simulink model "ASM_Traffic"  (R2026a)
settings: Solver=ode1  StartTime=SIM.tstart.v  StopTime=SIM.tend.v  FixedStep=SIM.StepSize.v
PostLoadFcn:
  | if any(exist('dsrtsu_mdlpostloadfcn', 'file') ~= 0), dsrtsu_mdlpostloadfcn('Execute', bdroot); end
  | try, asm_mdl_postloadfcn(bdroot, 'UpdateModel', 3600); catch, disp(lasterr); end,
InitFcn:
  | , if any(exist('rtifpga_mdlclblib', 'file') ~= 0), rtifpga_mdlclblib('Init', bdroot); end,
  | , if any(exist('dsmpb_private', 'file') ~= 0), dsmpb_private('dsmpb_mdlclblib', 'Init', bdroot); end,
model workspace (MAT data in the model file):
  asmReferencePath = [0 0.01 0.02 0.03 0.04 0.05 0.06 0.07 0.08 0.09 0.1 0.11 ... (350007 elements, 50001x7)]
  roadBounds : Simulink.Parameter (value not decoded)
  safetyAxes : Simulink.Parameter (value not decoded)
undefined symbols (not defined in the file): _to_, a0b2, ASM_BrakeHydraulics_DemoSystems, ASM_VehicleDynamics_DemoSystems, b98103fe8ad365046cd0, BrakeCircuit, controllerConfig, CPT, Crankshaft, DiscIntNeverNeededParam, dsmsi, FinalDriveAssembly, MDL, ModeSignals, mu, Pos_BrakePedal_Maneuver, rad, RefSignals, roadFamilyData, roadFamilyId, s_to_rpm, SIM, SoftECU, Suspension, Tire, Transmission
libraries: ASM_Traffic_lib x135, simulink x98, ASM_Utils_lib x77, ASM_VehicleDynamics_lib x70, ASM_Environment_lib x22, dsmpblib x20, dsmsilib x15, MDLD_Utils_lib x10, ASM_BrakeHydraulics_lib x3, sl_discontinuities x2
(part 28 of 65)

== system ASM_Traffic/Environment/Road/PlantModel/Pos_CP_CoorsSys_E[:][x;y][m] ==
  Pos_CP[x;y][m] : Inport
  Active_CP_VehDyn_Trailer[] : Inport  Port=2
  Bus Selector : BusSelector  OutputSignals=Pos_CP_FL_CoorSys_E[x;y][m],Pos_CP_FR_CoorSys_E[x;y][m],Pos_CP_RL_CoorSys_E[x;y][m],Pos_CP_RL2_CoorSys_E[x;y][m],Pos_CP_RR_CoorSys_E[x;y][m],Pos_CP_RR2_CoorSys_E[x;y][m],Pos_CP_R2L_CoorSys_E[x;y][m],Pos_CP_R2L2_CoorSys_E[x;y][m],Pos_CP_R2R_CoorSys_E[x;y][m],Pos_CP_R2R2_CoorSys_E[x;y][m],Pos_CP_FL_Trailer_CoorSys_E[x;y][m],Pos_CP_FL2_Trailer_CoorSys_E[x;y][m],Pos_CP_FR_Trailer_CoorSys_E[x;y][m],Pos_CP_FR2_Trailer_CoorSys_E[x;y][m],Pos_CP_RL_Trailer_CoorSys_E[x;y][m],Pos_CP_RL2_Trailer_CoorSys_E[x;y][m],Pos_CP_RR_Trailer_CoorSys_E[x;y][m],Pos_CP_RR2_Trailer_CoorSys_E[x;y][m],Pos_CP_R2L_Trailer_CoorSys_E[x;y][m],Pos_CP_R2L2_Trailer_CoorSys_E[x;y][m],Pos_CP_R2R_Trailer_CoorSys_E[x;y][m],Pos_CP_R2R2_Trailer_CoorSys_E[x;y][m],Pos_CP_Front_CoorSys_E[x;y][m],Pos_CP_Rear_CoorSys_E[x;y][m]
  Mux : Mux  Inputs=24
  Selector : Selector  IndexOptions=Index vector (port)  Indices=[1 3]  OutputSizes=1
  Pos_CP_CoorsSys_E[:][x;y][m] : Outport  VectorParamsAs1DForOutWhenUnconnected=off
  wires:
  Bus Selector/24 -> Mux/24  "<Pos_CP_Rear_CoorSys_E[x;y][m]>"
  Bus Selector/23 -> Mux/23  "<Pos_CP_Front_CoorSys_E[x;y][m]>"
  Selector/1 -> Pos_CP_CoorsSys_E[:][x;y][m]/1
  Active_CP_VehDyn_Trailer[]/1 -> Selector/2
  Pos_CP[x;y][m]/1 -> Bus Selector/1
  Bus Selector/1 -> Mux/1  "<Pos_CP_FL_CoorSys_E[x;y][m]>"
  Bus Selector/2 -> Mux/2  "<Pos_CP_FR_CoorSys_E[x;y][m]>"
  Bus Selector/3 -> Mux/3  "<Pos_CP_RL_CoorSys_E[x;y][m]>"
  Bus Selector/4 -> Mux/4  "<Pos_CP_RL2_CoorSys_E[x;y][m]>"
  Bus Selector/5 -> Mux/5  "<Pos_CP_RR_CoorSys_E[x;y][m]>"
  Bus Selector/6 -> Mux/6  "<Pos_CP_RR2_CoorSys_E[x;y][m]>"
  Bus Selector/7 -> Mux/7  "<Pos_CP_R2L_CoorSys_E[x;y][m]>"
  Bus Selector/8 -> Mux/8  "<Pos_CP_R2L2_CoorSys_E[x;y][m]>"
  Bus Selector/9 -> Mux/9  "<Pos_CP_R2R_CoorSys_E[x;y][m]>"
  Bus Selector/10 -> Mux/10  "<Pos_CP_R2R2_CoorSys_E[x;y][m]>"
  Bus Selector/11 -> Mux/11  "<Pos_CP_FL_Trailer_CoorSys_E[x;y][m]>"
  Bus Selector/12 -> Mux/12  "<Pos_CP_FL2_Trailer_CoorSys_E[x;y][m]>"
  Bus Selector/13 -> Mux/13  "<Pos_CP_FR_Trailer_CoorSys_E[x;y][m]>"
  Bus Selector/14 -> Mux/14  "<Pos_CP_FR2_Trailer_CoorSys_E[x;y][m]>"
  Bus Selector/15 -> Mux/15  "<Pos_CP_RL_Trailer_CoorSys_E[x;y][m]>"
  Bus Selector/16 -> Mux/16  "<Pos_CP_RL2_Trailer_CoorSys_E[x;y][m]>"
  Bus Selector/17 -> Mux/17  "<Pos_CP_RR_Trailer_CoorSys_E[x;y][m]>"
  Bus Selector/18 -> Mux/18  "<Pos_CP_RR2_Trailer_CoorSys_E[x;y][m]>"
  Bus Selector/19 -> Mux/19  "<Pos_CP_R2L_Trailer_CoorSys_E[x;y][m]>"
  Bus Selector/20 -> Mux/20  "<Pos_CP_R2L2_Trailer_CoorSys_E[x;y][m]>"
  Bus Selector/21 -> Mux/21  "<Pos_CP_R2R_Trailer_CoorSys_E[x;y][m]>"
  Bus Selector/22 -> Mux/22  "<Pos_CP_R2R2_Trailer_CoorSys_E[x;y][m]>"
  Mux/1 -> Selector/1

== system ASM_Traffic/Environment/Road/PlantModel/Reload_Trigger ==
  Init_External_Additional[0Off|1On] : Inport
  Interface_Mode[0Off|1ObjectsOnly|2ObjectsAndLanes] : Inport  Port=2
  Constant3 : Constant  Value=0.5
  Constant5 : Constant
  Constant6 : Constant  Value=0
  Logical Operator1 : Logic  AllPortsSameDT=off
  Relational Operator2 : RelationalOperator  Operator=>  OutDataTypeStr=boolean  InputSameDT=off
  Start : MultiPortSwitch  DataPortOrder=Zero-based contiguous  Inputs=2  zeroidx=on  InputSameDT=off
  Ctrl_Reload[] : Outport  VectorParamsAs1DForOutWhenUnconnected=off
  wires:
  Relational Operator2/1 -> Logical Operator1/1
  Constant3/1 -> Relational Operator2/2
  Init_External_Additional[0Off|1On]/1 -> Logical Operator1/2
  Logical Operator1/1 -> Start/1
  Interface_Mode[0Off|1ObjectsOnly|2ObjectsAndLanes]/1 -> Relational Operator2/1
  Start/1 -> Ctrl_Reload[]/1  "start"
  Constant5/1 -> Start/3
  Constant6/1 -> Start/2

== system ASM_Traffic/Environment/Road/UserInterface/ASMSignalBus_Plant ==
  In : Inport
  Terminator_1 : Terminator
  tag scope: ASMBUS_Environment_Road=global
  wires:
  [ASMBUS_Environment_Road] -> Terminator_1/1
  In/1 -> [ASMBUS_Environment_Road]

== system ASM_Traffic/Environment/Road/UserInterface/DISP_Plant ==
  In : Inport
  Ambient : Scope  NumInputPorts=2
      settings: TimeSpan=5  ActiveDisplayYMinimum=-0.4375  ActiveDisplayYMaximum=3.9375  DataLoggingMaxPoints=20000  DataLoggingDecimation=10
  Angle_Yaw_Veh_Road[deg] : Subsystem
      mask Display: disp('')
  BorderMode : Display
  Bus Selector : BusSelector  OutputSignals=Ambient.T_Ambient[degC],Ambient.p_Ambient[Pa]
  Bus Selector1 : BusSelector  OutputSignals=LaneSensor_Dynamic.Parameters.Border_Mode[0Center|1Inner|2Outer],LaneSensor_Dynamic.Sensor_Output.CurrentLane.Common.LaneWidth[m],LaneSensor_Dynamic.Sensor_Output.CurrentLane.LeftSide.MarkerType_Left[],LaneSensor_Dynamic.Sensor_Output.CurrentLane.RightSide.MarkerType_Right[],LaneSensor_Dynamic.Sensor_Output.CurrentLane.LeftSide.Distance_Marker_Left[m],LaneSensor_Dynamic.Sensor_Output.CurrentLane.RightSide.Distance_Marker_Right[m],LaneSensor_Dynamic.Sensor_Output.Measurement_Points.Distance_MeasPnt_Marker_Left[m],LaneSensor_Dynamic.Sensor_Output.Measurement_Points.Distance_MeasPnt_Marker_Right[m],LaneSensor_Dynamic.Sensor_Output.Measurement_Points.Velocity_MeasPnt_Marker_Left[m|s],LaneSensor_Dynamic.Sensor_Output.Measurement_Points.Velocity_MeasPnt_Marker_Right[m|s]
  Bus Selector2 : BusSelector  OutputSignals=Road_ASMVeh.Curv_Veh_Road[1|m],Road_ASMVeh.Slope_Veh_Road[%],Road_ContactPoints.Fric_Coeff_CP[:][],Road_ContactPoints.Pos_z_CP[:][m],Road_ContactPoints.Sw_Tire_Parameter_Set_CP[:][1|2|3|4],Road_ASMVeh.s_Veh_Road[m],Road_ASMVeh.Pos_x_Ref_Veh_Road[m],Road_ASMVeh.Pos_y_Ref_Veh_Road[m],Road_ASMVeh.Angle_Yaw_Veh_Road[deg],Pos_Vehicle_GPS[Long;Lat][deg].Longitude[deg],Pos_Vehicle_GPS[Long;Lat][deg].Latitude[deg]
  Curv_Veh_Road[1|m] : Subsystem
      mask Display: disp('')
  Distance_Marker_Left[m] : Subsystem
      mask Display: disp('')
  Distance_Marker_Right[m] : Subsystem
      mask Display: disp('')
  Distance_MeasPnt1_Marker_Left[m] : Subsystem
      mask Display: disp('')
  Distance_MeasPnt1_Marker_Right[m] : Subsystem
      mask Display: disp('')
  Distance_MeasPnt2_Marker_Left[m] : Subsystem
      mask Display: disp('')
  Distance_MeasPnt2_Marker_Right[m] : Subsystem
      mask Display: disp('')
  Fric_Coeff_CP[:][] : Subsystem
      mask Display: disp('')
  GPS_Latitude_Road[deg] : Subsystem
      mask Display: disp('')
  GPS_Longitude_Road[deg] : Subsystem
      mask Display: disp('')
  LaneSensorDynamic : Scope  NumInputPorts=5
      settings: TimeSpan=5  ActiveDisplayYMinimum=-0.4375  ActiveDisplayYMaximum=3.9375  DataLoggingMaxPoints=20000  DataLoggingDecimation=10
  LaneSensorDynamic_MeasPnts : Scope  NumInputPorts=8
      settings: TimeSpan=5  ActiveDisplayYMinimum=-2.74252  ActiveDisplayYMaximum=6.59287  DataLoggingMaxPoints=20000  DataLoggingDecimation=10  DataLoggingVariableName=ScopeData2
  LaneWidth[m] : Subsystem
      mask Display: disp('')
  MarkerType_Left[] : Subsystem
      mask Display: disp('')
  MarkerType_Right[] : Subsystem
      mask Display: disp('')
  Pos_x_Ref_Veh_Road[m] : Subsystem
      mask Display: disp('')
  Pos_y_Ref_Veh_Road[m] : Subsystem
      mask Display: disp('')
  Pos_z_CP[:][m] : Subsystem
      mask Display: disp('')
  RoadOverview : Scope  NumInputPorts=5
      settings: TimeSpan=5  ActiveDisplayYMinimum=-1  ActiveDisplayYMaximum=1  DataLoggingMaxPoints=20000  DataLoggingDecimation=10  DataLoggingVariableName=ScopeData3
  RoadPositions : Scope  NumInputPorts=6
      settings: TimeSpan=5  ActiveDisplayYMinimum=-23.27391  ActiveDisplayYMaximum=209.46515  DataLoggingMaxPoints=20000  DataLoggingDecimation=10  DataLoggingVariableName=ScopeData4
  Selector{,1,4..5} (4 alike) : Selector  IndexOptions=Index vector (dialog)  Indices=[1]  OutputSizes=1
  Selector{2..3,6..7} (4 alike) : Selector  IndexOptions=Index vector (dialog)  Indices=[2]  OutputSizes=1
  Slope_Veh_Road[%] : Subsystem
      mask Display: disp('')
  Sw_Tire_Parameter_Set_CP[:][1|2|3|4] : Subsystem
      mask Display: disp('')
  T_Ambient[degC] : Subsystem
      mask Display: disp('')
  Velocity_MeasPnt1_Marker_Left[m|s] : Subsystem
      mask Display: disp('')
  Velocity_MeasPnt1_Marker_Right[m|s] : Subsystem
      mask Display: disp('')
  Velocity_MeasPnt2_Marker_Left[m|s] : Subsystem
      mask Display: disp('')
  Velocity_MeasPnt2_Marker_Right[m|s] : Subsystem
      mask Display: disp('')
  p_Ambient[Pa] : Subsystem
      mask Display: disp('')
  s_Veh_Road[m] : Subsystem
      mask Display: disp('')
  wires:
  Bus Selector/2 -> p_Ambient[Pa]/1(In1)  "<p_Ambient[Pa]>"
  Bus Selector/1 -> T_Ambient[degC]/1(In1)  "<T_Ambient[degC]>"
  p_Ambient[Pa]/1(Out1) -> Ambient/2  "p_Ambient[Pa]"
  T_Ambient[degC]/1(Out1) -> Ambient/1  "T_Ambient[degC]"
  Bus Selector2/5 -> Sw_Tire_Parameter_Set_CP[:][1|2|3|4]/1(In1)  "<Sw_Tire_Parameter_Set_CP[:][1|2|3|4]>"
  Bus Selector2/11 -> GPS_Latitude_Road[deg]/1(In1)  "<Latitude[deg]>"
  Curv_Veh_Road[1|m]/1(Out1) -> RoadOverview/1  "Curv_Veh_Road[1|m]"
  Bus Selector2/8 -> Pos_y_Ref_Veh_Road[m]/1(In1)  "<Pos_y_Ref_Veh_Road[m]>"
  Bus Selector2/10 -> GPS_Longitude_Road[deg]/1(In1)  "<Longitude[deg]>"
  Bus Selector2/1 -> Curv_Veh_Road[1|m]/1(In1)  "<Curv_Veh_Road[1|m]>"
  Sw_Tire_Parameter_Set_CP[:][1|2|3|4]/1(Out1) -> RoadOverview/5  "Sw_Tire_Parameter_Set_CP[:][1|2|3|4]"
  Pos_z_CP[:][m]/1(Out1) -> RoadOverview/4  "Pos_z_CP[:][m]"
  Bus Selector2/7 -> Pos_x_Ref_Veh_Road[m]/1(In1)  "<Pos_x_Ref_Veh_Road[m]>"
  Bus Selector2/4 -> Pos_z_CP[:][m]/1(In1)  "<Pos_z_CP[:][m]>"
  Bus Selector2/2 -> Slope_Veh_Road[%]/1(In1)  "<Slope_Veh_Road[%]>"
  Fric_Coeff_CP[:][]/1(Out1) -> RoadOverview/3  "Fric_Coeff_CP[:][]"
  In/1 -> Bus Selector/1, Bus Selector1/1, Bus Selector2/1
  GPS_Longitude_Road[deg]/1(Out1) -> RoadPositions/5  "GPS_Longitude_Road[deg]"
  Bus Selector1/5 -> Distance_Marker_Left[m]/1(In1)  "<Distance_Marker_Left[m]>"
  Bus Selector1/1 -> BorderMode/1  "<Border_Mode[0Center|1Inner|2Outer]>"
  Distance_Marker_Right[m]/1(Out1) -> LaneSensorDynamic/5  "Distance_Marker_Right[m]"
  Bus Selector1/9 -> Selector3/1, Selector1/1  "<Velocity_MeasPnt_Marker_Left[m|s]>"
  Bus Selector2/3 -> Fric_Coeff_CP[:][]/1(In1)  "<Fric_Coeff_CP[:][]>"
  Bus Selector1/10 -> Selector7/1, Selector5/1  "<Velocity_MeasPnt_Marker_Right[m|s]>"
  s_Veh_Road[m]/1(Out1) -> RoadPositions/1  "s_Veh_Road[m]"
  Bus Selector2/9 -> Angle_Yaw_Veh_Road[deg]/1(In1)  "<Angle_Yaw_Veh_Road[deg]>"
  Bus Selector1/8 -> Selector6/1, Selector4/1  "<Distance_MeasPnt_Marker_Right[m]>"
  Distance_MeasPnt1_Marker_Left[m]/1(Out1) -> LaneSensorDynamic_MeasPnts/1  "Distance_MeasPnt1_Marker_Left[m]"
  Slope_Veh_Road[%]/1(Out1) -> RoadOverview/2  "Slope_Veh_Road[%]"
  Bus Selector2/6 -> s_Veh_Road[m]/1(In1)  "<s_Veh_Road[m]>"
  Selector7/1 -> Velocity_MeasPnt2_Marker_Right[m|s]/1(In1)
  Angle_Yaw_Veh_Road[deg]/1(Out1) -> RoadPositions/4  "Angle_Yaw_Veh_Road[deg]"
  Selector4/1 -> Distance_MeasPnt1_Marker_Right[m]/1(In1)
  Velocity_MeasPnt1_Marker_Left[m|s]/1(Out1) -> LaneSensorDynamic_MeasPnts/3  "Velocity_MeasPnt1_Marker_Left[m|s]"
  Bus Selector1/4 -> MarkerType_Right[]/1(In1)  "<MarkerType_Right[]>"
  Bus Selector1/3 -> MarkerType_Left[]/1(In1)  "<MarkerType_Left[]>"
  Velocity_MeasPnt2_Marker_Right[m|s]/1(Out1) -> LaneSensorDynamic_MeasPnts/8  "Velocity_MeasPnt2_Marker_Right[m|s]"
  Velocity_MeasPnt2_Marker_Left[m|s]/1(Out1) -> LaneSensorDynamic_MeasPnts/7  "Velocity_MeasPnt2_Marker_Left[m|s]"
  Distance_MeasPnt1_Marker_Right[m]/1(Out1) -> LaneSensorDynamic_MeasPnts/2  "Distance_MeasPnt1_Marker_Right[m]"
  Bus Selector1/2 -> LaneWidth[m]/1(In1)  "<LaneWidth[m]>"
  Bus Selector1/6 -> Distance_Marker_Right[m]/1(In1)  "<Distance_Marker_Right[m]>"
  Distance_MeasPnt2_Marker_Right[m]/1(Out1) -> LaneSensorDynamic_MeasPnts/6  "Distance_MeasPnt2_Marker_Right[m]"
  Bus Selector1/7 -> Selector2/1, Selector/1  "<Distance_MeasPnt_Marker_Left[m]>"
  LaneWidth[m]/1(Out1) -> LaneSensorDynamic/1  "LaneWidth[m]"
  Distance_MeasPnt2_Marker_Left[m]/1(Out1) -> LaneSensorDynamic_MeasPnts/5  "Distance_MeasPnt2_Marker_Left[m]"
  MarkerType_Left[]/1(Out1) -> LaneSensorDynamic/2  "MarkerType_Left[]"
  GPS_Latitude_Road[deg]/1(Out1) -> RoadPositions/6  "GPS_Latitude_Road[deg]"
  Selector6/1 -> Distance_MeasPnt2_Marker_Right[m]/1(In1)
  Selector/1 -> Distance_MeasPnt1_Marker_Left[m]/1(In1)
  Distance_Marker_Left[m]/1(Out1) -> LaneSensorDynamic/4  "Distance_Marker_Left[m]"
  Selector5/1 -> Velocity_MeasPnt1_Marker_Right[m|s]/1(In1)
  Selector2/1 -> Distance_MeasPnt2_Marker_Left[m]/1(In1)
  Velocity_MeasPnt1_Marker_Right[m|s]/1(Out1) -> LaneSensorDynamic_MeasPnts/4  "Velocity_MeasPnt1_Marker_Right[m|s]"
  Selector1/1 -> Velocity_MeasPnt1_Marker_Left[m|s]/1(In1)
  Pos_y_Ref_Veh_Road[m]/1(Out1) -> RoadPositions/3  "Pos_y_Ref_Veh_Road[m]"
  Pos_x_Ref_Veh_Road[m]/1(Out1) -> RoadPositions/2  "Pos_x_Ref_Veh_Road[m]"
  MarkerType_Right[]/1(Out1) -> LaneSensorDynamic/3  "MarkerType_Right[]"
  Selector3/1 -> Velocity_MeasPnt2_Marker_Left[m|s]/1(In1)

== system ASM_Traffic/Environment/Road/UserInterface/PAR_Plant ==
  note: Control
  note: Inport colors:
  note: -------------
  note: Plant
  note: External Signals
  note: -------------
  note: -------------
  note: -------------
  note: User Interface
  Interface_In : Inport
  BasicRoad : Subsystem
      mask Display: disp('Basic Road')
  Bus Creator : BusCreator  Inputs=3
  Bus Selector1 : BusSelector  OutputSignals=Interface_In.ExternalModel.Active_CP_VehDyn_Trailer[]
  Bus Selector2 : BusSelector  OutputSignals=Interface_In.ExternalModel.Pos_CP_FL_CoorSys_E[x;y][m],Interface_In.ExternalModel.Pos_CP_FR_CoorSys_E[x;y][m],Interface_In.ExternalModel.Pos_CP_RL_CoorSys_E[x;y][m],Interface_In.ExternalModel.Pos_CP_RL2_CoorSys_E[x;y][m],Interface_In.ExternalModel.Pos_CP_RR_CoorSys_E[x;y][m],Interface_In.ExternalModel.Pos_CP_RR2_CoorSys_E[x;y][m],Interface_In.ExternalModel.Pos_CP_R2L_CoorSys_E[x;y][m],Interface_In.ExternalModel.Pos_CP_R2L2_CoorSys_E[x;y][m],Interface_In.ExternalModel.Pos_CP_R2R_CoorSys_E[x;y][m],Interface_In.ExternalModel.Pos_CP_R2R2_CoorSys_E[x;y][m],Interface_In.ExternalModel.Pos_CP_FL_Trailer_CoorSys_E[x;y][m],Interface_In.ExternalModel.Pos_CP_FL2_Trailer_CoorSys_E[x;y][m],Interface_In.ExternalModel.Pos_CP_FR_Trailer_CoorSys_E[x;y][m],Interface_In.ExternalModel.Pos_CP_FR2_Trailer_CoorSys_E[x;y][m],Interface_In.ExternalModel.Pos_CP_RL_Trailer_CoorSys_E[x;y][m],Interface_In.ExternalModel.Pos_CP_RL2_Trailer_CoorSys_E[x;y][m],Interface_In.ExternalModel.Pos_CP_RR_Trailer_CoorSys_E[x;y][m],Interface_In.ExternalModel.Pos_CP_RR2_Trailer_CoorSys_E[x;y][m],Interface_In.ExternalModel.Pos_CP_R2L_Trailer_CoorSys_E[x;y][m],Interface_In.ExternalModel.Pos_CP_R2L2_Trailer_CoorSys_E[x;y][m],Interface_In.ExternalModel.Pos_CP_R2R_Trailer_CoorSys_E[x;y][m],Interface_In.ExternalModel.Pos_CP_R2R2_Trailer_CoorSys_E[x;y][m],Interface_In.ExternalModel.Pos_CP_Front_CoorSys_E[x;y][m],Interface_In.ExternalModel.Pos_CP_Rear_CoorSys_E[x;y][m]  OutputAsBus=on
  Bus Selector4 : BusSelector  OutputSignals=Maneuver.Plant.ManeuverScheduler.Info.ManeuverState[],Maneuver.Plant.UserSignals_Customized.Mnv_DataStream_5[],Maneuver.Plant.UserSignals_Customized.Mnv_DataStream_6[],Maneuver.Plant.UserSignals_Customized.Mnv_DataStream_7[],Maneuver.Plant.UserSignals_Customized.Mnv_DataStream_8[]  OutputAsBus=on
  Objects_DataStreams : Subsystem
      mask Display: disp('Objects Data Streams')
  Pos_CP_CoorsSys_E[:][x;y][m] : Subsystem
  ROAD_SELECT_SWITCH : ASM_Environment_lib/Environment/Road/ROAD_SELECT_SWITCH  Tag=ASM_SUBCOMPONENT  SW_Road_Select=MDL.Environment.SW_Road_Select.v  ASMProperties=struct('Name','ROAD_SELECT_SWITCH','Version','2.0','Library','ASM_Environment_lib')  ASMInstanceName=road_select_switch  ASMInstanceID=1
  Out : Outport  VectorParamsAs1DForOutWhenUnconnected=off
  wires:
  Objects_DataStreams/1(Out1) -> Bus Creator/3
  Bus Selector4/1 -> Objects_DataStreams/1(In1)
  ROAD_SELECT_SWITCH/1 -> Bus Creator/1  "Sw_RoadSelect[1_6]"
  BasicRoad/1(Out1) -> Bus Creator/2
  Bus Creator/1 -> Out/1  "UserInterface"
  Interface_In/1 -> Bus Selector2/1, Bus Selector1/1, Bus Selector4/1
  Bus Selector1/1 -> Pos_CP_CoorsSys_E[:][x;y][m]/2(Active_CP_VehDyn_Trailer[])  "<Active_CP_VehDyn_Trailer[]>"
  Bus Selector2/1 -> Pos_CP_CoorsSys_E[:][x;y][m]/1(Pos_CP[x;y][m])
  Pos_CP_CoorsSys_E[:][x;y][m]/1(Pos_CP_CoorsSys_E[:][x;y][m]) -> BasicRoad/1(Pos_CP_CoorSys_E[:][x;y][m])

== system ASM_Traffic/Environment/Sensors/PlantModel/ASMSignalCollector ==
  Bus Creator1 : BusCreator  Inputs=6
  Sensors : Outport  VectorParamsAs1DForOutWhenUnconnected=off
  wires:
  [ASMBUS_Environment_Traffic_Sensors_Collision_Sensor] -> Bus Creator1/5
  [ASMBUS_Environment_Traffic_Sensors_Line_Sensor] -> Bus Creator1/4
  [ASMBUS_Environment_Traffic_Sensors_Common] -> Bus Creator1/6
  [ASMBUS_Environment_Traffic_Sensors_Object_Sensor_2D] -> Bus Creator1/2
  Bus Creator1/1 -> Sensors/1  "Sensors"
  [ASMBUS_Environment_Trafffic_Sensors_Object_Sensor_3D] -> Bus Creator1/1
  [ASMBUS_Environment_Traffic_Sensors_Traffic_Sign_Sensor_dyn] -> Bus Creator1/3

== system ASM_Traffic/Environment/Sensors/PlantModel/Collision_Sensor ==
  Enable_Init[0Off|1On] : Inport
  Enable[0Off|1On] : Inport  Port=2
  Traffic_Signals : Inport  Port=3
  Interface_In : Inport  Port=4
  Road_Signals : Inport  Port=5
  Maneuver_Signals : Inport  Port=6
  ASMSignalCollector : Subsystem
  Bus Selector : BusSelector  OutputSignals=Plant.Traffic_Signals_toEnvironment.v_Fellows[x;y;z][km|h],Plant.Traffic_Signals_toEnvironment.w_Fellows[x;y;z][deg|s]
  Bus Selector1 : BusSelector  OutputSignals=ExternalModel.Pos_Vehicle_CoorSys_E[x;y;z][m],ExternalModel.Angle_Vehicle_CoorSys_E[x;y;z][deg],ExternalModel.v_x_Vehicle_CoG[km|h],ExternalModel.v_y_Vehicle_CoG[km|h],ExternalModel.YawRate_Vehicle_CoG[deg|s]
  Bus Selector2 : BusSelector  OutputSignals=Plant.ObjectParameters.FellowParameters.TrafficObject_Type_Fellows[],Plant.ObjectParameters.TrafficObjects.TrafficObject_Type_Data[],Plant.ObjectParameters.DiscreteObjects.DiscreteObject_Data[]
  Bus Selector3 : BusSelector  OutputSignals=Plant.TrafficObject_Data[]
  Bus Selector4 : BusSelector  OutputSignals=Plant.Traffic_Signals_toEnvironment
  Bus Selector5 : BusSelector  OutputSignals=Plant.ManeuverScheduler.Info.ManeuverTime[s],Plant.ManeuverScheduler.Parameters.Object_Type_ID[]
  Bus Selector6 : BusSelector  OutputSignals=Info.Flag_Sensor_Init_Ready[0|1]  OutputAsBus=on
  Bus Selector7 : BusSelector  OutputSignals=Plant.Traffic_Signals_toEnvironment.Flag_FellowUsed[0|1]
  Bus Selector8 : BusSelector  OutputSignals=Plant.ObjectParameters.TrafficObjects.TrafficObjectsState[],Plant.ObjectParameters.DiscreteObjects.DiscreteObjectsState[]
  COLLISION_SENSOR : ASM_Traffic_lib/Sensors/Collision_Sensor/COLLISION_SENSOR  Tag=ASM_SUBCOMPONENT  Sw_Sensor_Enable=MDL.Traffic.Sensors.CollisionSensor.Sw_Sensor_Enable  Sw_Detection_Mode=MDL.Traffic.Sensors.CollisionSensor.Sw_Detection_Mode  Const_Collisions_OutputDimension=MDL.Traffic.Sensors.CollisionSensor.Const_Sensor_Output_Dimension  ASMProperties=struct('Name','COLLISION_SENSOR','Version','5.0','Library','ASM_Traffic_lib')  ASMInstanceName=collision_sensor  ASMInstanceID=1
  Constant : Constant  Value=0
  Demux : Demux  Outputs=3
  Enable_Collision_Sensor : Subsystem
  ExternalUserData : Subsystem
  GetFellowPositionVector : Subsystem
  Mux : Mux  Inputs=3
  Mux1 : Mux  Inputs=2
  Mux2 : Mux  Inputs=2
  SensorsGotoTagVisiblity : GotoTagVisibility  GotoTag=ASMBUS_Traf_Sensors_Collision_Sensor_1
  Terminator : Terminator
  Terminator2 : Terminator
  Terminator3 : Terminator
  Sensor_Signals : Outport  VectorParamsAs1DForOutWhenUnconnected=off
  tag scope: ASMBUS_Traf_Sensors_Collision_Sensor_1=scoped
  wires:
  Bus Selector7/1 -> COLLISION_SENSOR/9  "<Flag_FellowUsed[0|1]>"
  GetFellowPositionVector/2(Angle_Fellows[deg]) -> COLLISION_SENSOR/11
  GetFellowPositionVector/1(Pos_Fellows_MainPnt_CoorSys_E[x;y;z][m]) -> COLLISION_SENSOR/10
  Bus Selector4/1 -> GetFellowPositionVector/1(<FellowPositions>)  "<Traffic_Signals_toEnvironment>"
  Bus Selector6/1 -> Terminator3/1
  COLLISION_SENSOR/2 -> Bus Selector6/1, Sensor_Signals/1
  Enable_Init[0Off|1On]/1 -> COLLISION_SENSOR/1
  ExternalUserData/1(Flag_CollsionSensor_Parameters_Used_External[0|1]) -> COLLISION_SENSOR/14
  ExternalUserData/4(Pos_y_CollisionObj_Custom_RefPnt_External[m]) -> Mux1/2
  ExternalUserData/3(Pos_x_CollisionObj_Custom_RefPnt_External[m]) -> Mux1/1
  Bus Selector/1 -> COLLISION_SENSOR/12  "<v_Fellows[x;y;z][km|h]>"
  Bus Selector/2 -> Demux/1  "<w_Fellows[x;y;z][deg|s]>"
  Demux/3 -> COLLISION_SENSOR/13
  Demux/1 -> Terminator/1
  Demux/2 -> Terminator2/1
  Constant/1 -> Mux/3
  Bus Selector5/1 -> COLLISION_SENSOR/7  "<ManeuverTime[s]>"
  Bus Selector5/2 -> COLLISION_SENSOR/8  "<Object_Type_ID[]>"
  Maneuver_Signals/1 -> Bus Selector5/1
  Mux/1 -> COLLISION_SENSOR/5
  COLLISION_SENSOR/1 -> [ASMBUS_Traf_Sensors_Collision_Sensor_1]
  Bus Selector3/1 -> COLLISION_SENSOR/20  "<TrafficObject_Data[]>"
  Bus Selector2/3 -> COLLISION_SENSOR/19  "<DiscreteObject_Data[]>"
  Bus Selector2/2 -> COLLISION_SENSOR/18  "<TrafficObject_Type_Data[]>"
  Bus Selector2/1 -> COLLISION_SENSOR/17  "<TrafficObject_Type_Fellows[]>"
  Mux1/1 -> COLLISION_SENSOR/16
  ExternalUserData/2(TrafficObject_Type_CollisionObj_External[]) -> COLLISION_SENSOR/15
  Bus Selector1/5 -> COLLISION_SENSOR/6  "<YawRate_Vehicle_CoG[deg|s]>"
  Bus Selector1/4 -> Mux/2  "<v_y_Vehicle_CoG[km|h]>"
  Bus Selector1/3 -> Mux/1  "<v_x_Vehicle_CoG[km|h]>"
  Bus Selector1/2 -> COLLISION_SENSOR/4  "<Angle_Vehicle_CoorSys_E[x;y;z][deg]>"
  Bus Selector1/1 -> COLLISION_SENSOR/3  "<Pos_Vehicle_CoorSys_E[x;y;z][m]>"
  Enable_Collision_Sensor/1(Enable_Out[0Off|1On]) -> COLLISION_SENSOR/2
  Enable[0Off|1On]/1 -> Enable_Collision_Sensor/1(Enable_In[0Off|1On])
  Interface_In/1 -> Bus Selector1/1
  Road_Signals/1 -> Bus Selector3/1
  Bus Selector8/2 -> Mux2/2  "<DiscreteObjectsState[]>"
  Mux2/1 -> COLLISION_SENSOR/21
  Bus Selector8/1 -> Mux2/1  "<TrafficObjectsState[]>"
  Traffic_Signals/1 -> Bus Selector7/1, Bus Selector4/1, Bus Selector2/1, Bus Selector8/1, Bus Selector/1

== system ASM_Traffic/Environment/Sensors/PlantModel/Line_Sensor ==
  Enable[0Off|1On] : Inport
  Interface_In : Inport  Port=2
  Road_Signals : Inport  Port=3
  Maneuver_Signals : Inport  Port=4
  ASMSignalCollector : Subsystem
  Bus Selector15 : BusSelector  OutputSignals=ExternalModel.Pos_Vehicle_CoorSys_E[x;y;z][m],ExternalModel.Angle_Vehicle_CoorSys_E[x;y;z][deg]
  Bus Selector2 : BusSelector  OutputSignals=Plant.Road_Info.Line_Sensor_Data
  Bus Selector5 : BusSelector  OutputSignals=Plant.ManeuverScheduler.MdlControl.Reset_VehicleStates[0|1],Plant.ManeuverScheduler.Info.ManeuverState[],Plant.ManeuverScheduler.InitialVehStates.Route_Id_Init[],Plant.ManeuverScheduler.InitialVehStates.Route_Direction_Init[]
  Bus Selector6 : BusSelector  OutputSignals=Plant.Road_ASMVeh.s_Veh_Road[m],Plant.Road_Info.d_Veh_Ref_Line[m]
  Demux : Demux  Outputs=3
  Demux1 : Demux  Outputs=3
  Enable_Line_Sensor : Subsystem
  LINE_SENSOR : ASM_Traffic_lib/Sensors/Line_Sensor/LINE_SENSOR  Tag=ASM_SUBCOMPONENT  Const_Length_Sensor_Range=MDL.Traffic.Sensors.LineSensor.Const_Length_Sensor_Range  Const_Num_Lines_Per_Side_Max=MDL.Traffic.Sensors.LineSensor.Const_Num_Lines_Per_Side_Max  Const_Dist_Road_Sample_Pnts=MDL.Traffic.Sensors.LineSensor.Const_Dist_Road_Sample_Pnts  Const_Road_Lane_Output_Dimension=MDL.Traffic.Sensors.LineSensor.Const_Road_Lane_Output_Dimension  Const_Road_Shape_Line_Output_Dimension=MDL.Traffic.Sensors.LineSensor.Const_Road_Shape_Line_Output_Dimension  Const_Road_Shape_ContObj_Output_Dimension=MDL.Traffic.Sensors.LineSensor.Const_Road_Shape_ContObj_Output_Dimension  Const_Junction_Border_Output_Dimension=MDL.Traffic.Sensors.LineSensor.Const_Junction_Border_Output_Dimension  Const_Junction_Shape_Line_Output_Dimension=MDL.Traffic.Sensors.LineSensor.Const_Junction_Shape_Line_Output_Dimension  Const_Junction_Shape_ContObj_Output_Dimension=MDL.Traffic.Sensors.LineSensor.Const_Junction_Shape_ContObj_Output_Dimension  Sw_Sensor_Enable=MDL.Traffic.Sensors.LineSensor.Sw_Sensor_Enable  ASMProperties=struct('Name','LINE_SENSOR','Version','8.0','Library','ASM_Traffic_lib')  ASMInstanceName=line_sensor  ASMInstanceID=1
  SensorsGotoTagVisiblity : GotoTagVisibility  GotoTag=ASMBUS_Traf_Sensors_Line_Sensor_1
  Terminator17 : Terminator
  Terminator18 : Terminator
  Terminator19 : Terminator
  Sensor_Signals : Outport  VectorParamsAs1DForOutWhenUnconnected=off
  tag scope: ASMBUS_Traf_Sensors_Line_Sensor_1=scoped
  wires:
  Enable_Line_Sensor/1(Enable_Out[0Off|1On]) -> LINE_SENSOR/1
  Bus Selector6/2 -> LINE_SENSOR/8  "<d_Veh_Ref_Line[m]>"
  Interface_In/1 -> Bus Selector15/1
  Bus Selector6/1 -> LINE_SENSOR/7  "<s_Veh_Road[m]>"
  Road_Signals/1 -> Bus Selector2/1, Bus Selector6/1
  Bus Selector5/4 -> LINE_SENSOR/6  "<Route_Direction_Init[]>"
  Bus Selector5/3 -> LINE_SENSOR/5  "<Route_Id_Init[]>"
  Bus Selector5/2 -> LINE_SENSOR/4  "<ManeuverState[]>"
  Bus Selector5/1 -> LINE_SENSOR/3  "<Reset_VehicleStates[0|1]>"
  Maneuver_Signals/1 -> Bus Selector5/1
  Enable[0Off|1On]/1 -> Enable_Line_Sensor/1(Enable_In[0Off|1On])
  Bus Selector2/1 -> LINE_SENSOR/2  "<Line_Sensor_Data>"
  LINE_SENSOR/2 -> Sensor_Signals/1
  LINE_SENSOR/1 -> [ASMBUS_Traf_Sensors_Line_Sensor_1]
  Demux/1 -> Terminator19/1
  Demux1/3 -> Terminator18/1
  Bus Selector15/2 -> Demux/1  "<Angle_Vehicle_CoorSys_E[x;y;z][deg]>"
  Demux/2 -> Terminator17/1
  Bus Selector15/1 -> Demux1/1  "<Pos_Vehicle_CoorSys_E[x;y;z][m]>"
  Demux1/1 -> LINE_SENSOR/9
  Demux1/2 -> LINE_SENSOR/10
  Demux/3 -> LINE_SENSOR/11

== system ASM_Traffic/Environment/Sensors/PlantModel/Object_Sensor_2D ==
  Enable_Init[0Off|1On] : Inport
  Enable[0Off|1On] : Inport  Port=2
  Traffic_Signals : Inport  Port=3
  Interface_In : Inport  Port=4
  Road_Signals : Inport  Port=5
  ASMSignalCollector : Subsystem
  Enable_Object_Sensor_2D : Subsystem
  ObjectData : Subsystem
  ScheduleAndCalculateSensor : Subsystem
  SensorMapping : Subsystem
  SensorParameters : Subsystem
  SensorsGotoTagVisiblity1 : GotoTagVisibility  GotoTag=ASMBUS_Environment_Traffic_2DObjSensor_ObjectData
  SensorsGotoTagVisiblity2 : GotoTagVisibility  GotoTag=ASMBUS_Environment_Traffic_SensorScheduler_ObjectSensor2D
  SensorsGotoTagVisiblity3 : GotoTagVisibility  GotoTag=ASMBUS_Environment_Traffic_2DObjSensor_Parameter
  SensorsGotoTagVisiblity4 : GotoTagVisibility  GotoTag=ASMBUS_Environment_Traffic_2DObjSensorCalc_Info
  SensorsGotoTagVisiblity5 : GotoTagVisibility  GotoTag=ASMBUS_Environment_Traffic_2DObjSensor_SensorSignals
  SensorsGotoTagVisiblity6 : GotoTagVisibility  GotoTag=ASMBUS_Environment_Traffic_SamplePulse_ObjectSensor2D
  Sensor_Signals : Outport  VectorParamsAs1DForOutWhenUnconnected=off
  Init_Ready[0Off|1On] : Outport  Port=2  VectorParamsAs1DForOutWhenUnconnected=off
  wires:
  ScheduleAndCalculateSensor/3(Init_Ready[0Off|1On]) -> Init_Ready[0Off|1On]/1
  Enable_Init[0Off|1On]/1 -> ScheduleAndCalculateSensor/1(Enable_Init[0Off|1On])
  Enable[0Off|1On]/1 -> Enable_Object_Sensor_2D/1(Enable_In[0Off|1On])
  Enable_Object_Sensor_2D/1(Enable_Out[0Off|1On]) -> SensorMapping/1(Enable[0Off|1On]), ScheduleAndCalculateSensor/3(Enable[0Off|1On])
  SensorMapping/1(Sensor_Signals) -> Sensor_Signals/1
  Interface_In/1 -> ScheduleAndCalculateSensor/5(Interface_In)
  Traffic_Signals/1 -> ScheduleAndCalculateSensor/4(Traffic_Signals), ObjectData/1(Traffic_Signals)
  Road_Signals/1 -> ScheduleAndCalculateSensor/6(Road_Signals), ObjectData/2(Road_Signals)
  ScheduleAndCalculateSensor/1(SensorMapping_Data[]) -> SensorMapping/2(SensorMapping_Data[])
  ScheduleAndCalculateSensor/2(SensorSignals) -> SensorMapping/3(SensorSignals)
  SensorParameters/1(Sensor_Data[]) -> ScheduleAndCalculateSensor/2(Sensor_Data[])

== system ASM_Traffic/Environment/Sensors/PlantModel/Object_Sensor_3D ==
  Enable_Init[0Off|1On] : Inport
  Enable[0Off|1On] : Inport  Port=2
  Traffic_Signals : Inport  Port=3
  Interface_In : Inport  Port=4
  Road_Signals : Inport  Port=5
  Sensor_Time_Base[s] : Inport  Port=6
  ASMSignalCollector : Subsystem
  CustomPoints : Subsystem
  Enable_Object_Sensor_3D : Subsystem
  ObjectData : Subsystem
  RadarEffects : Subsystem
  ScheduleAndCalculateSensor : Subsystem
  SensorMapping : Subsystem
  SensorParameters : Subsystem
  SensorsGotoTagVisiblity1 : GotoTagVisibility  GotoTag=ASMBUS_Environment_Traffic_3DObjSensor_CustomPoints
  SensorsGotoTagVisiblity10 : GotoTagVisibility  GotoTag=ASMBUS_Environment_Traffic_3DObjSensor2_Parameters
  SensorsGotoTagVisiblity11 : GotoTagVisibility  GotoTag=ASMBUS_Environment_Traffic_3DObjSensor3_Parameters
  SensorsGotoTagVisiblity2 : GotoTagVisibility  GotoTag=ASMBUS_Environment_Traffic_3DObjSensors_Boundingboxes
  SensorsGotoTagVisiblity3 : GotoTagVisibility  GotoTag=ASMBUS_Environment_Traffic_3DObjSensor_ObjectData
  SensorsGotoTagVisiblity4 : GotoTagVisibility  GotoTag=ASMBUS_Environment_Traffic_3DObjSensor_RadarEffects
  SensorsGotoTagVisiblity5 : GotoTagVisibility  GotoTag=ASMBUS_Environment_Traffic_SensorScheduler
  SensorsGotoTagVisiblity6 : GotoTagVisibility  GotoTag=ASMBUS_Environment_Traffic_SamplePulse
  SensorsGotoTagVisiblity7 : GotoTagVisibility  GotoTag=ASMBUS_Environment_Traffic_3DObjSensor_SensorSignals_Status
  SensorsGotoTagVisiblity8 : GotoTagVisibility  GotoTag=ASMBUS_Environment_Traffic_3DObjSensor_SensorSignals
  SensorsGotoTagVisiblity9 : GotoTagVisibility  GotoTag=ASMBUS_Environment_Traffic_3DObjSensor1_Parameters
  Sensor_Signals : Outport  VectorParamsAs1DForOutWhenUnconnected=off
  Init_Ready[0Off|1On] : Outport  Port=2  VectorParamsAs1DForOutWhenUnconnected=off
  wires:
  ScheduleAndCalculateSensor/3(SensorData[]) -> RadarEffects/4(SensorData[]), CustomPoints/3(SensorData[])
  ScheduleAndCalculateSensor/4(Angle_Vehicle_CoorSys_E_Sampled[x,y;z][deg]) -> RadarEffects/5(Angle_Vehicle_CoorSys_E[x;y;z][deg])
  ScheduleAndCalculateSensor/5(Pos_Vehicle_CoorSys_E_Sampled[x,y;z][m]) -> RadarEffects/6(Pos_Vehicle_CoorSys_E[x;y;z][m])
  Enable_Init[0Off|1On]/1 -> ScheduleAndCalculateSensor/1(Enable_Init[0Off|1On]), RadarEffects/1(Enable_Init[0Off|1On])
  ScheduleAndCalculateSensor/6(Init_Ready[0Off|1On]) -> Init_Ready[0Off|1On]/1
  Enable[0Off|1On]/1 -> Enable_Object_Sensor_3D/1(Enable_In[0Off|1On])
  Enable_Object_Sensor_3D/1(Enable_Out[0Off|1On]) -> ScheduleAndCalculateSensor/3(Enable[0Off|1On]), CustomPoints/1(Enable[0Off|1On]), RadarEffects/2(Enable[0Off|1On]), SensorMapping/1(Enable[0Off|1On])
  SensorMapping/1(Sensor_Signals) -> Sensor_Signals/1
  Interface_In/1 -> ScheduleAndCalculateSensor/5(Interface_In)
  SensorParameters/1(Sensor_Data[]) -> ScheduleAndCalculateSensor/2(Sensor_Data[])
  Traffic_Signals/1 -> ObjectData/1(Traffic_Signals), ScheduleAndCalculateSensor/4(Traffic_Signals)
  Road_Signals/1 -> ObjectData/2(Road_Signals), ScheduleAndCalculateSensor/6(Road_Signals)
  ScheduleAndCalculateSensor/1(SensorMapping_Data[]) -> CustomPoints/2(SensorMapping_Data[]), RadarEffects/3(SensorMapping_Data[]), SensorMapping/2(SensorMapping_Data[])
  ScheduleAndCalculateSensor/2(SensorSignals) -> SensorMapping/3(SensorSignals)
  Sensor_Time_Base[s]/1 -> ScheduleAndCalculateSensor/7(Sensor_Time_Base[s])

== system ASM_Traffic/Environment/Sensors/PlantModel/Sensors_Common_Signals ==
  In : Inport
  Init_Ready[0Off|1On] : Inport  Port=2
  Brake : RelationalOperator  Operator===  OutDataTypeStr=boolean  InputSameDT=off
  Bus Selector2 : BusSelector  OutputSignals=Traffic.Plant.ObjectParameters.DiscreteObjects.Flag_DiscreteObject_Init_Ready[0|1]
  Bus Selector7 : BusSelector  OutputSignals=Maneuver.Plant.ManeuverScheduler.Info.ManeuverState[]  OutputAsBus=on
  Constant : Constant  Value=3
  Constant1 : Constant  Value=4
  Data Type Conversion : DataTypeConversion  OutDataTypeStr=double  SaturateOnIntegerOverflow=off  RndMeth=Floor
  Enable_Scheduling : Subsystem
  Logical Operator : Logic  Operator=OR  AllPortsSameDT=off  OutDataTypeStr=boolean
  Logical Operator1 : Logic  AllPortsSameDT=off
  Maneuver_Start : Subsystem
  Memory : UnitDelay  SampleTime=-1
  Run : RelationalOperator  Operator===  OutDataTypeStr=boolean  InputSameDT=off
  Sensor_Init_Trigger : Subsystem
  Sensor_Time_Base : Subsystem
  SignalCollector : Subsystem
  ASMSignalBus : Outport  VectorParamsAs1DForOutWhenUnconnected=off
  Enable_Init[0Off|1On] : Outport  Port=2  VectorParamsAs1DForOutWhenUnconnected=off
  Enable_Sensor_Scheduling_By_Init_Ready[0Off|1On] : Outport  Port=3  VectorParamsAs1DForOutWhenUnconnected=off
  Enable_Sensor_Scheduling[0Off|1On] : Outport  Port=4  VectorParamsAs1DForOutWhenUnconnected=off
  Sensor_Time_Base[s] : Outport  Port=5
  wires:
  Bus Selector2/1 -> Sensor_Init_Trigger/1(DiscreteObjects_Data_Valid[])  "<Flag_DiscreteObject_Init_Ready[0|1]>"
  Sensor_Init_Trigger/1(Ctrl) -> Enable_Init[0Off|1On]/1
  Init_Ready[0Off|1On]/1 -> Memory/1, SignalCollector/3(Init_Ready[0Off|1On])
  Memory/1 -> Logical Operator1/1
  Logical Operator1/1 -> Enable_Sensor_Scheduling_By_Init_Ready[0Off|1On]/1
  Enable_Scheduling/1(Enable_Out[0Off|1On]) -> Logical Operator1/2, Enable_Sensor_Scheduling[0Off|1On]/1
  Data Type Conversion/1 -> Enable_Scheduling/1(Enable_In[0Off|1On]), SignalCollector/2(Enable_SensorScheduling[0Off|1On])
  SignalCollector/1(ASMSignalBus) -> ASMSignalBus/1
  Brake/1 -> Logical Operator/2
  Bus Selector7/1 -> Brake/1, Run/1
  Constant1/1 -> Brake/2
  Run/1 -> Logical Operator/1
  Constant/1 -> Run/2
  Maneuver_Start/1(ManeuverStart[s]) -> Sensor_Time_Base/2(ManeuverStart[s]), SignalCollector/1(ManeuverStart[s])
  In/1 -> Bus Selector2/1, Bus Selector7/1
  Logical Operator/1 -> Sensor_Time_Base/1(ManeuverState_Change[0|1]), Maneuver_Start/1(ManeuverState_Change[0|1]), Data Type Conversion/1
  Sensor_Time_Base/1(Sensor_Time_Base[s]) -> Sensor_Time_Base[s]/1

== system ASM_Traffic/Environment/Sensors/PlantModel/Traffic_Sign_Sensor ==
  Interface_In : Inport
  Traffic_Signals : Inport  Port=2
  Road_Signals : Inport  Port=3
  Objects_DataStream_Signals : Inport  Port=4
  ASMSignalCollector : Subsystem
  Bus Selector1 : BusSelector  OutputSignals=ExternalModel.Pos_Vehicle_CoorSys_E[x;y;z][m],ExternalModel.Angle_Vehicle_CoorSys_E[x;y;z][deg]
  Bus Selector2 : BusSelector  OutputSignals=Plant.ObjectParameters.TrafficObjects.TrafficObject_Type_Data[]
  Bus Selector3 : BusSelector  OutputSignals=Plant.TrafficObject_Data[]
  Enable_Traffic_Sign_Sensor : Subsystem
  Mux : Mux  Inputs=6
  Objects_DataStreams : Subsystem
  SensorsGotoTagVisiblity : GotoTagVisibility  GotoTag=ASMBUS_Traf_Sensors_Traffic_Sign_Sensor_dyn_1_Parameters
  SensorsGotoTagVisiblity1 : GotoTagVisibility  GotoTag=ASMBUS_Traf_Sensors_dyn_Traffic_Sign_Sensor_1
  TRAFFIC_SIGN_SENSOR_DYNAMIC_CALCULATION : ASM_Traffic_lib/Sensors/Traffic_Sign_Sensor/TRAFFIC_SIGN_SENSOR_DYNAMIC_CALCULATION  Tag=ASM_SUBCOMPONENT  Const_Sensor_Output_Dimension=MDL.Traffic.Sensors.TrafficSignSensorDyn_Calculation.Const_Sensor_Output_Dimension  ASMProperties=struct('Name','TRAFFIC_SIGN_SENSOR_DYNAMIC_CALCULATION','Version','2.0','Library','ASM_Traffic_lib')  ASMInstanceName=traffic_sign_sensor_dynamic_calculation  ASMInstanceID=1
  TRAFFIC_SIGN_SENSOR_GEOMETRY_PARAMETERS : ASM_Traffic_lib/Sensors/Traffic_Sign_Sensor/TRAFFIC_SIGN_SENSOR_GEOMETRY_PARAMETERS  Tag=ASM_SUBCOMPONENT  Sensor_Enable=MDL.Traffic.Sensors.TrafficSignSensor_Geometry.Sw_Sensor_Enable  Pos_Sensor=MDL.Traffic.Sensors.TrafficSignSensor_Geometry.Const_Pos_Sensor_Apex_CoorSys_V  Angle_Orientation_Sensor=MDL.Traffic.Sensors.TrafficSignSensor_Geometry.Const_Angle_Orientation_Sensor_CoorSys_V  Length_ScopeZone=MDL.Traffic.Sensors.TrafficSignSensor_Geometry.Const_Length_ScopeZone  Angle_ScopeZone_Horizontal=MDL.Traffic.Sensors.TrafficSignSensor_Geometry.Const_Angle_ScopeZone_Horizontal  Angle_ScopeZone_Vertical=MDL.Traffic.Sensors.TrafficSignSensor_Geometry.Const_Angle_ScopeZone_Vertical  Angle_Sign_Orientation_Max=MDL.Traffic.Sensors.TrafficSignSensor_Geometry.Const_Angle_Sign_Orientation_Max  ASMProperties=struct('Name','TRAFFIC_SIGN_SENSOR_GEOMETRY_PARAMETERS','Version','2.0','Library','ASM_Traffic_lib')  ASMInstanceName=traffic_sign_sensor_geometry_parameters  ASMInstanceID=1
  Sensor_Signals : Outport  VectorParamsAs1DForOutWhenUnconnected=off
  tag scope: ASMBUS_Traf_Sensors_Traffic_Sign_Sensor_dyn_1_Parameters=scoped, ASMBUS_Traf_Sensors_dyn_Traffic_Sign_Sensor_1=scoped
  wires:
  Objects_DataStream_Signals/1 -> Objects_DataStreams/1(TrafficObjects_States_In[])
  Objects_DataStreams/1(TrafficObjects_States[]) -> TRAFFIC_SIGN_SENSOR_DYNAMIC_CALCULATION/7
  Bus Selector3/1 -> TRAFFIC_SIGN_SENSOR_DYNAMIC_CALCULATION/6  "<TrafficObject_Data[]>"
  Bus Selector2/1 -> TRAFFIC_SIGN_SENSOR_DYNAMIC_CALCULATION/5  "<TrafficObject_Type_Data[]>"
  Bus Selector1/2 -> TRAFFIC_SIGN_SENSOR_DYNAMIC_CALCULATION/4  "<Angle_Vehicle_CoorSys_E[x;y;z][deg]>"
  Bus Selector1/1 -> TRAFFIC_SIGN_SENSOR_DYNAMIC_CALCULATION/3  "<Pos_Vehicle_CoorSys_E[x;y;z][m]>"
  TRAFFIC_SIGN_SENSOR_DYNAMIC_CALCULATION/2 -> Sensor_Signals/1
  TRAFFIC_SIGN_SENSOR_DYNAMIC_CALCULATION/1 -> [ASMBUS_Traf_Sensors_dyn_Traffic_Sign_Sensor_1]
  Enable_Traffic_Sign_Sensor/1(Enable_Out[0Off|1On]) -> TRAFFIC_SIGN_SENSOR_DYNAMIC_CALCULATION/1
  TRAFFIC_SIGN_SENSOR_GEOMETRY_PARAMETERS/1 -> [ASMBUS_Traf_Sensors_Traffic_Sign_Sensor_dyn_1_Parameters]
  TRAFFIC_SIGN_SENSOR_GEOMETRY_PARAMETERS/2 -> Enable_Traffic_Sign_Sensor/1(Enable_In[0Off|1On])
  Mux/1 -> TRAFFIC_SIGN_SENSOR_DYNAMIC_CALCULATION/2
  TRAFFIC_SIGN_SENSOR_GEOMETRY_PARAMETERS/8 -> Mux/6
  TRAFFIC_SIGN_SENSOR_GEOMETRY_PARAMETERS/7 -> Mux/5
  TRAFFIC_SIGN_SENSOR_GEOMETRY_PARAMETERS/6 -> Mux/4
  TRAFFIC_SIGN_SENSOR_GEOMETRY_PARAMETERS/5 -> Mux/3
  TRAFFIC_SIGN_SENSOR_GEOMETRY_PARAMETERS/4 -> Mux/2
  TRAFFIC_SIGN_SENSOR_GEOMETRY_PARAMETERS/3 -> Mux/1
  Road_Signals/1 -> Bus Selector3/1
  Traffic_Signals/1 -> Bus Selector2/1
  Interface_In/1 -> Bus Selector1/1

== system ASM_Traffic/Environment/Sensors/UserInterface/ASMSignalBus_Plant ==
  In : Inport
  Terminator_1 : Terminator
  tag scope: ASMBUS_Environment_Traffic_Sensors=global
  wires:
  In/1 -> [ASMBUS_Environment_Traffic_Sensors]
  [ASMBUS_Environment_Traffic_Sensors] -> Terminator_1/1

== system ASM_Traffic/Environment/Sensors/UserInterface/DISP_Plant ==
  In : Inport
  Line_Sensor : Subsystem
  Object_Sensor_2D : Subsystem
  Object_Sensor_3D : Subsystem
  Traffic_Sign_Sensor : Subsystem
  wires:
  In/1 -> Line_Sensor/1(TrafficBus), Traffic_Sign_Sensor/1(TrafficBus), Object_Sensor_2D/1(TrafficBus), Object_Sensor_3D/1(TrafficBus)

== system ASM_Traffic/Environment/Sensors/UserInterface/PAR_Plant ==
  note: Control
  note: Inport colors:
  note: -------------
  note: Plant
  note: External Signals
  note: -------------
  note: -------------
  note: -------------
  note: User Interface
  In : Inport
  Constant : Constant
  Terminator1 : Terminator
  Out : Outport  VectorParamsAs1DForOutWhenUnconnected=off
  wires:
  Constant/1 -> Out/1  "UserInterface"
  In/1 -> Terminator1/1
